simulink model "all_sb2_0001_0004"  (R2026a)
settings: Solver=VariableStepAuto  StopTime=24.0
settings Model: Creator=ldy  LastModifiedBy=harry_31916

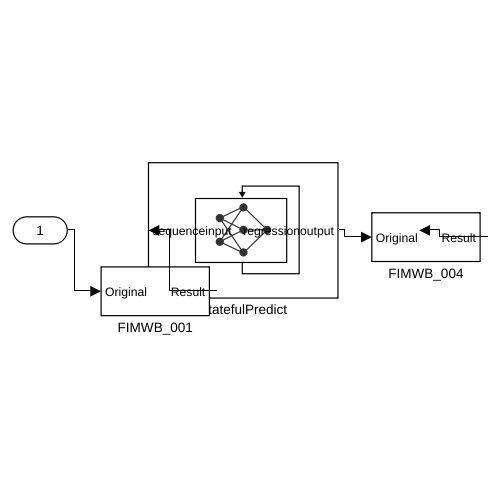
[thumbnail: Simulink's stored preview of the top-level diagram]
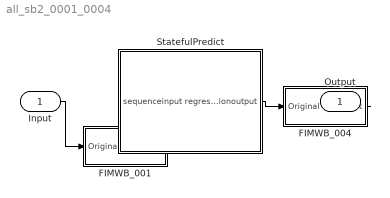
== system all_sb2_0001_0004 ==
  Input : Inport
  FIMWB_001 : Subsystem  Tag=fimwb.fault.1
  FIMWB_004 : Subsystem  Tag=fimwb.fault.4
  StatefulPredict : Subsystem  mask(Stateful Predict){Network=Network from MAT-file, NetworkFunction=untitled, NetworkFilePath=phi2_m1_vr01_k2_2.mat, SimulateUsing=Auto mode, InputDataFormats={'',''}, SampleTime=1, ForceInterpretedSim=off, EnableDLNetwork=on, LastKnownNetworkFilePath='', LastKnownNetworkTimeStamp=''}
      mask prompts: Network "deep_blocks:common:Network"; NetworkFunction "deep_blocks:common:MatlabFunction"; NetworkFilePath "deep_blocks:common:FilePath"; SimulateUsing "Simulate using:"; InputDataFormats "deep_blocks:predict:InputDataFormats"; SampleTime "deep_blocks:common:SampleTime"; ForceInterpretedSim "deep_blocks:common:ForceInterpretedSim"
      mask help: deep_blocks:stateful:PredictDescription
      mask init:
      | deep.blocks.internal.configureSequenceNetworkPredict(...
      |     gcb, ...
      |     bdroot, ...
      |     Network, ...
      |     NetworkFilePath, ...
      |     NetworkFunction, ...
      |     InputDataFormats, ...
      |     logical(ForceInterpretedSim), ...
      |     SimulateUsing);
      mask Help: helpview('deeplearning', 'nnet_stateful_predict')
      mask TypeOptions Network: deep_blocks:common:NetworkFromMatFile | deep_blocks:common:NetworkFromFunction
      mask Callback Network:
      | deep.blocks.internal.setNetworkSelectVisibility(gcb);
      | deep.blocks.internal.setDlNetworkOptionsVisibility(gcb);
      mask Callback NetworkFunction: deep.blocks.internal.setDlNetworkOptionsVisibility(gcb);
      mask Callback NetworkFilePath: deep.blocks.internal.setDlNetworkOptionsVisibility(gcb);
      mask TypeOptions SimulateUsing: deep_blocks:common:SimModeAuto | deep_blocks:common:SimModeInterpreted | deep_blocks:common:SimModeCodegen
      mask DialogControl Network Prompt: Network:
      mask DialogControl NetworkFunction Prompt: MATLAB function:
      mask DialogControl NetworkFilePath Prompt: File path:
      mask DialogControl BrowseButton Prompt: deep_blocks:common:Browse
      mask DialogControl BrowseButton Callback: deep.blocks.internal.handleBrowseButtonClick(gcb);
      mask DialogControl SimulateUsing Tooltip: deep_blocks:common:SimModeTooltip
      mask DialogControl InputDataFormats Prompt: Input data formats:
      mask DialogControl SampleTime Prompt: Sample time (-1 for inherited):
      mask DialogControl HiddenContainer Prompt: Hidden Parameters
      mask DialogControl ForceInterpretedSim Prompt: Force interpreted simulation
  Output : Outport
  wires:
  Input/1 -> FIMWB_001/1(Original)
  FIMWB_001/1(Result) -> StatefulPredict/1(sequenceinput)
  StatefulPredict/1(regressionoutput) -> FIMWB_004/1(Original)
  FIMWB_004/1(Result) -> Output/1

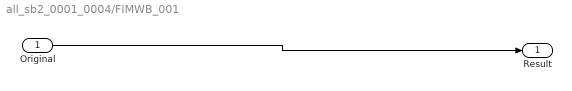
== system all_sb2_0001_0004/FIMWB_001 ==
  Original : Inport
  Result : Outport
  wires:
  Original/1 -> Result/1

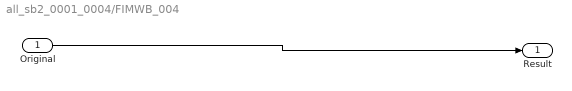
== system all_sb2_0001_0004/FIMWB_004 ==
  Original : Inport
  Result : Outport
  wires:
  Original/1 -> Result/1

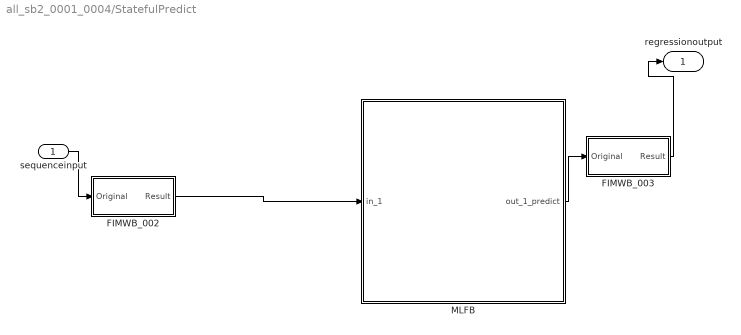
== system all_sb2_0001_0004/StatefulPredict ==
  sequenceinput : Inport
  FIMWB_002 : Subsystem  Tag=fimwb.fault.2
  FIMWB_003 : Subsystem  Tag=fimwb.fault.3
  MLFB : MATLAB Function  TreatAsAtomicUnit=on
  regressionoutput : Outport
  wires:
  sequenceinput/1 -> FIMWB_002/1(Original)
  FIMWB_002/1(Result) -> MLFB/1(in_1)
  MLFB/1(out_1_predict) -> FIMWB_003/1(Original)
  FIMWB_003/1(Result) -> regressionoutput/1

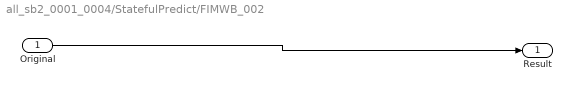
== system all_sb2_0001_0004/StatefulPredict/FIMWB_002 ==
  Original : Inport
  Result : Outport
  wires:
  Original/1 -> Result/1

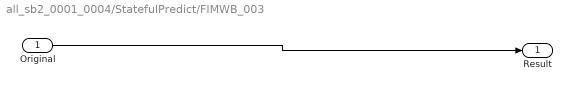
== system all_sb2_0001_0004/StatefulPredict/FIMWB_003 ==
  Original : Inport
  Result : Outport
  wires:
  Original/1 -> Result/1

== matlab function all_sb2_0001_0004/StatefulPredict/MLFB ==
  settings: updateMethod=DISCRETE  sampleTime=1
  data: in_1 input; out_1_predict output
function out_1_predict  = sequenceNetworkPredict( in_1 )
isSim = coder.target('sfun');
simSupported = false;
useExtrinsic = isSim && ~simSupported;
[out_1_predict] = deep.blocks.internal.sequenceNetworkPredict({in_1}, {size(in_1)}, {class(in_1)}, coder.const("all_sb2_0001_0004/StatefulPredict"), 'phi2_m1_vr01_k2_2.mat', useExtrinsic, false, 1, {''});
end
